simulink model "r2_b16a4x64f"  (R2012b)
settings: Solver=VariableStepDiscrete  SolverMode=SingleTasking  StartTime=0.0  StopTime=1  RelTol=1e-3
undefined symbols (not defined in the file): fft_stages, n_bits_ants, n_bits_xengs
libraries: xbsIndex_r4 x26846, casper_library_misc x230, xbsReplacements_r4 x24, casper_library_delays x8, xps_library x5, casper_library_communications x4
(part 46 of 227)

== system r2_b16a4x64f/sys2/Delay89 ==
  d : Inport
  Register0 : xbsIndex_r4/Register  init=0  rst=off  en=off  dbl_ovrd=off  block_type=register
      settings: block_version=11.4
  Register1 : xbsIndex_r4/Register  init=0  rst=off  en=off  dbl_ovrd=off  block_type=register
  q : Outport
  wires:
  Register0/1 -> Register1/1
  d/1 -> Register0/1
  Register1/1 -> q/1

== system r2_b16a4x64f/sys2/Delay9 ==
  d : Inport
  Register0 : xbsIndex_r4/Register  init=0  rst=off  en=off  dbl_ovrd=off  block_type=register
      settings: block_version=11.4
  Register1 : xbsIndex_r4/Register  init=0  rst=off  en=off  dbl_ovrd=off  block_type=register
  q : Outport
  wires:
  Register0/1 -> Register1/1
  d/1 -> Register0/1
  Register1/1 -> q/1

== system r2_b16a4x64f/sys2/bf ==
  synci : Inport
  di : Inport  Port=2
  deni : Inport  Port=3
  badi : Inport  Port=4
  timei : Inport  Port=5
  misci : Inport  Port=6
  beng_id : Inport  Port=7
  Delay1 : xbsIndex_r4/Delay  rst=off  infoeditControl=Selection of Reset will increase slice count due to use of real FFs and instead of SRLs  en=off  latency=1  dbl_ovrd=off  reg_retiming=on  block_type=delay
  Delay2 : xbsIndex_r4/Delay  rst=off  infoeditControl=Selection of Reset will increase slice count due to use of real FFs and instead of SRLs  en=off  latency=1  dbl_ovrd=off  reg_retiming=on  block_type=delay
  Relational : xbsIndex_r4/Relational  mode=a=b  en=off  latency=1  dbl_ovrd=off  block_type=relational
  Slice : xbsIndex_r4/Slice  nbits=bfpga_bits  boolean_output=off  mode=Lower Bit Location + Width  bit1=0  base1=MSB of Input  bit0=0  base0=LSB of Input  dbl_ovrd=off  block_type=slice
  fbf : Subsystem  mask(fbf){beng_bits=beng_bits, ant_bits=ant_bits, polarisation_bits=polarisation_bits, freq_bits=freq_bits, stack_bits=stack_bits, n_bits_in=n_bits_in, bin_pt_in=bin_pt_in, timestamp_bits=timestamp_bits, n_bits_norm=n_bits_norm, bin_pt_norm=bin_pt_norm, n_bits_combine=n_bits_combine, n_bits_requant=n_bits_requant, bin_pt_requant=bin_pt_requant, bram_latency=bram_latency, add_latency=add_latency, mult_latency=mult_latency, beam_bits=beam_bits, n_bits_out=n_bits_out, bin_pt_out=bin_pt_out, conv_latency=conv_latency, output_enabled=off}
      mask prompts: beng_bits "b-engines (2^?)"; ant_bits "antennas (2^?)"; polarisation_bits "polarisations (2^?)"; freq_bits "frequencies (2^?)"; stack_bits "stacking factor (2^?)"; n_bits_in "data bits in"; bin_pt_in "binary point in"; timestamp_bits "timestamp size (bits)"; n_bits_norm "calibration factor data bits"; bin_pt_norm "calibration factor binary point"; n_bits_combine "antenna combination output bit width"; n_bits_requant "requantization factor bit width"; bin_pt_requant "requantization factor binary point"; bram_latency "bram latency"; add_latency "add latency"; beam_bits "beams (2^?)"; n_bits_out "data bits out"; bin_pt_out "binary point out"; conv_latency "convert latency"; output_enabled "output enabled by default?"
      mask help:
      | Frequency domain beamformer
      |
      | b-engines: number of b-engines in system (same as x-engines)
      | stacking factor: the number of consecutive time samples in a data block
      | calibration factor: the complex factor multiplied with the incoming data.
      | The complex value is unique to each beam, input and frequency.
      | Requantization factor: real factor multiplied with the output data before
      | quantization. The value is unique to each beam and frequency.
      | beams: the number of beams per polarisation
      | ouput enabled by default: can be useful for simulation
      mask init:
      | set_param([gcb,'/filter'], ...
      |     'output_enabled', output_enabled);
      mask Help:
      | Accepts the same channelised data as the CASPER FX correlator x-engine core.
      | Polarisations appear in order in different beams. (for polarisation (0,1), 0 in [0,2...], 1 in [1,3...]).
      | TODO: beam steering.
      | TODO: Stokes output.
      | TODO: accumulation.
  synco : Outport
  do : Outport  Port=2
  deno : Outport  Port=3
  timeo : Outport  Port=4
  misco : Outport  Port=5
  value_out_bw : Outport  Port=6
  value_out_quant : Outport  Port=7
  value_out_filt : Outport  Port=8
  wires:
  fbf/3(deno) -> deno/1
  di/1 -> fbf/2(di)
  timei/1 -> fbf/5(timei)
  fbf/1(synco) -> synco/1
  [bf_stream] -> Delay2/1
  fbf/2(do) -> do/1
  misci/1 -> fbf/6(misci)
  synci/1 -> fbf/1(synci)
  deni/1 -> fbf/3(deni)
  [bf_antenna] -> Delay1/1
  badi/1 -> fbf/4(badi)
  fbf/4(timeo) -> timeo/1
  fbf/5(misco) -> misco/1
  fbf/6(bw_value_out) -> value_out_bw/1
  beng_id/1 -> Slice/1
  [bf_beng] -> Relational/2
  Slice/1 -> Relational/1
  Relational/1 -> fbf/9(ld_wr_en)
  Delay1/1 -> fbf/7(ld_antenna)
  Delay2/1 -> fbf/8(ld_stream)
  fbf/7(quant_value_out) -> value_out_quant/1
  fbf/8(filter_value_out) -> value_out_filt/1

== system r2_b16a4x64f/sys2/bus_expand1 ==
  bus_in : Inport
  reinterpret1 : xbsIndex_r4/Reinterpret  force_arith_type=on  arith_type=Unsigned  force_bin_pt=on  bin_pt=0  block_type=reinterpret
      settings: infoedit="Changes signal type without altering the binary representation.   You can changed the signal between signed and unsigned, and relocate the binary point.<br><br>Hardware notes: In hardware this block costs nothing.<br><br>Example:  Suppose the input is 6 bits wide, signed, with 2 fractional bits, and the output is forced to unsigned with 0 fractional bits.  Then an input of -2.0 (1110.00 in binary 2's complement) becomes an output of 56 (111000 in binary)."
  reinterpret3 : xbsIndex_r4/Reinterpret  force_arith_type=on  arith_type=Unsigned  force_bin_pt=on  bin_pt=0  block_type=reinterpret
  slice1 : xbsIndex_r4/Slice  nbits=32  boolean_output=off  mode=Upper Bit Location + Width  bit1=-28  base1=MSB of Input  bit0=0  base0=LSB of Input  dbl_ovrd=off  block_type=slice
  slice2 : xbsIndex_r4/Slice  nbits=1  boolean_output=on  mode=Upper Bit Location + Width  bit1=-27  base1=MSB of Input  bit0=0  base0=LSB of Input  dbl_ovrd=off  block_type=slice
  slice3 : xbsIndex_r4/Slice  nbits=27  boolean_output=off  mode=Upper Bit Location + Width  bit1=0  base1=MSB of Input  bit0=0  base0=LSB of Input  dbl_ovrd=off  block_type=slice
  msb_out3 : Outport
  out2 : Outport  Port=2
  lsb_out1 : Outport  Port=3
  wires:
  bus_in/1 -> slice3/1, slice2/1, slice1/1
  slice3/1 -> reinterpret3/1
  reinterpret3/1 -> msb_out3/1
  slice2/1 -> out2/1
  slice1/1 -> reinterpret1/1
  reinterpret1/1 -> lsb_out1/1

== system r2_b16a4x64f/sys2/bus_expand2 ==
  bus_in : Inport
  reinterpret1 : xbsIndex_r4/Reinterpret  force_arith_type=on  arith_type=Unsigned  force_bin_pt=on  bin_pt=0  block_type=reinterpret
  reinterpret2 : xbsIndex_r4/Reinterpret  force_arith_type=on  arith_type=Unsigned  force_bin_pt=on  bin_pt=0  block_type=reinterpret
  slice1 : xbsIndex_r4/Slice  nbits=19  boolean_output=off  mode=Upper Bit Location + Width  bit1=-27  base1=MSB of Input  bit0=0  base0=LSB of Input  dbl_ovrd=off  block_type=slice
  slice2 : xbsIndex_r4/Slice  nbits=27  boolean_output=off  mode=Upper Bit Location + Width  bit1=0  base1=MSB of Input  bit0=0  base0=LSB of Input  dbl_ovrd=off  block_type=slice
  msb_out2 : Outport
  lsb_out1 : Outport  Port=2
  wires:
  bus_in/1 -> slice2/1, slice1/1
  slice2/1 -> reinterpret2/1
  reinterpret2/1 -> msb_out2/1
  slice1/1 -> reinterpret1/1
  reinterpret1/1 -> lsb_out1/1

== system r2_b16a4x64f/sys2/bus_expand20 ==
  bus_in : Inport
  reinterpret1 : xbsIndex_r4/Reinterpret  force_arith_type=on  arith_type=Unsigned  force_bin_pt=on  bin_pt=0  block_type=reinterpret
      settings: infoedit="Changes signal type without altering the binary representation.   You can changed the signal between signed and unsigned, and relocate the binary point.<br><br>Hardware notes: In hardware this block costs nothing.<br><br>Example:  Suppose the input is 6 bits wide, signed, with 2 fractional bits, and the output is forced to unsigned with 0 fractional bits.  Then an input of -2.0 (1110.00 in binary 2's complement) becomes an output of 56 (111000 in binary)."
  reinterpret2 : xbsIndex_r4/Reinterpret  force_arith_type=on  arith_type=Unsigned  force_bin_pt=on  bin_pt=0  block_type=reinterpret
      settings: infoedit="Changes signal type without altering the binary representation.   You can changed the signal between signed and unsigned, and relocate the binary point.<br><br>Hardware notes: In hardware this block costs nothing.<br><br>Example:  Suppose the input is 6 bits wide, signed, with 2 fractional bits, and the output is forced to unsigned with 0 fractional bits.  Then an input of -2.0 (1110.00 in binary 2's complement) becomes an output of 56 (111000 in binary)."
  slice1 : xbsIndex_r4/Slice  nbits=19  boolean_output=off  mode=Upper Bit Location + Width  bit1=-33  base1=MSB of Input  bit0=0  base0=LSB of Input  dbl_ovrd=off  block_type=slice
  slice2 : xbsIndex_r4/Slice  nbits=33  boolean_output=off  mode=Upper Bit Location + Width  bit1=0  base1=MSB of Input  bit0=0  base0=LSB of Input  dbl_ovrd=off  block_type=slice
  msb_out2 : Outport
  lsb_out1 : Outport  Port=2
  wires:
  bus_in/1 -> slice2/1, slice1/1
  slice2/1 -> reinterpret2/1
  reinterpret2/1 -> msb_out2/1
  slice1/1 -> reinterpret1/1
  reinterpret1/1 -> lsb_out1/1

== system r2_b16a4x64f/sys2/bus_expand3 ==
  bus_in : Inport
  slice1 : xbsIndex_r4/Slice  nbits=1  boolean_output=on  mode=Upper Bit Location + Width  bit1=-5  base1=MSB of Input  bit0=0  base0=LSB of Input  dbl_ovrd=off  block_type=slice
  slice2 : xbsIndex_r4/Slice  nbits=1  boolean_output=on  mode=Upper Bit Location + Width  bit1=-4  base1=MSB of Input  bit0=0  base0=LSB of Input  dbl_ovrd=off  block_type=slice
  slice3 : xbsIndex_r4/Slice  nbits=1  boolean_output=on  mode=Upper Bit Location + Width  bit1=-3  base1=MSB of Input  bit0=0  base0=LSB of Input  dbl_ovrd=off  block_type=slice
  slice4 : xbsIndex_r4/Slice  nbits=1  boolean_output=on  mode=Upper Bit Location + Width  bit1=-2  base1=MSB of Input  bit0=0  base0=LSB of Input  dbl_ovrd=off  block_type=slice
  slice5 : xbsIndex_r4/Slice  nbits=1  boolean_output=on  mode=Upper Bit Location + Width  bit1=-1  base1=MSB of Input  bit0=0  base0=LSB of Input  dbl_ovrd=off  block_type=slice
  slice6 : xbsIndex_r4/Slice  nbits=1  boolean_output=on  mode=Upper Bit Location + Width  bit1=0  base1=MSB of Input  bit0=0  base0=LSB of Input  dbl_ovrd=off  block_type=slice
  msb_out6 : Outport
  out5 : Outport  Port=2
  out4 : Outport  Port=3
  out3 : Outport  Port=4
  out2 : Outport  Port=5
  lsb_out1 : Outport  Port=6
  wires:
  bus_in/1 -> slice6/1, slice5/1, slice4/1, slice3/1, slice2/1, slice1/1
  slice6/1 -> msb_out6/1
  slice5/1 -> out5/1
  slice4/1 -> out4/1
  slice3/1 -> out3/1
  slice2/1 -> out2/1
  slice1/1 -> lsb_out1/1

== system r2_b16a4x64f/sys2/bus_relational ==
  a : Inport
  b : Inport  Port=2
  a_debus : Subsystem  AncestorBlock=casper_library_flow_control/bus_expand  mask(bus_expand){mode=divisions of arbitrary size, outputNum=1, outputWidth=[1  1  1  1  1  1  1  1  1  1  1  1  1  1  1  1  1  1  1], outputBinaryPt=[0  0  0  0  0  0  0  0  0  0  0  0  0  0  0  0  0  0  0], outputArithmeticType=[0  0  0  0  0  0  0  0  0  0  0  0  0  0  0  0  0  0  0], show_format=on, outputToWorkspace=off, variablePrefix=, outputToModelAsWell=on}
      mask prompts: outputNum "Number of outputs:"; outputWidth "Output width [msb ... lsb]:"; outputBinaryPt "Output binary point position [msb ... lsb]:"; outputArithmeticType "Output arithmetic type (ufix=0, fix=1, bool=2) [msb ... lsb]:"; show_format "Print format string?"; outputToWorkspace "Output to workspace?"; variablePrefix "Variable name prefix:"; outputToModelAsWell "Output to model as well?"
      mask help:
      | Expands a 'bus' made using a bus_create or Xilinx
      | concat block.
      | The input will be divided into the specified number
      | of outputs with the specified arithmetic types.
      | Divisions are made from most significant bit.
      mask init: same as r2_b16a4x64f/bus_expand
      settings: AttributesFormatString=19 outputs: uf1.0,uf1.0,uf1.0,uf1.0,uf1.0,uf1.0,uf1.0,uf1.0,uf1.0,uf1.0,uf1.0,uf1.0,uf1.0,uf1.0,uf1.0,uf1.0,uf1.0,uf1.0,uf1.0,
      mask TypeOptions mode: divisions of equal size | divisions of arbitrary size
      mask Callback mode: bus_expand_callback();
      mask Callback outputWidth: bus_expand_callback();
      mask Callback outputToWorkspace: bus_expand_callback();
  b_debus : Subsystem  AncestorBlock=casper_library_flow_control/bus_expand  mask(bus_expand){mode=divisions of arbitrary size, outputNum=1, outputWidth=[1  1  1  1  1  1  1  1  1  1  1  1  1  1  1  1  1  1  1], outputBinaryPt=[0  0  0  0  0  0  0  0  0  0  0  0  0  0  0  0  0  0  0], outputArithmeticType=[0  0  0  0  0  0  0  0  0  0  0  0  0  0  0  0  0  0  0], show_format=on, outputToWorkspace=off, variablePrefix=, outputToModelAsWell=on}
      mask prompts: outputNum "Number of outputs:"; outputWidth "Output width [msb ... lsb]:"; outputBinaryPt "Output binary point position [msb ... lsb]:"; outputArithmeticType "Output arithmetic type (ufix=0, fix=1, bool=2) [msb ... lsb]:"; show_format "Print format string?"; outputToWorkspace "Output to workspace?"; variablePrefix "Variable name prefix:"; outputToModelAsWell "Output to model as well?"
      mask help:
      | Expands a 'bus' made using a bus_create or Xilinx
      | concat block.
      | The input will be divided into the specified number
      | of outputs with the specified arithmetic types.
      | Divisions are made from most significant bit.
      mask init: same as r2_b16a4x64f/bus_expand
      settings: AttributesFormatString=19 outputs: uf1.0,uf1.0,uf1.0,uf1.0,uf1.0,uf1.0,uf1.0,uf1.0,uf1.0,uf1.0,uf1.0,uf1.0,uf1.0,uf1.0,uf1.0,uf1.0,uf1.0,uf1.0,uf1.0,
      mask TypeOptions mode: divisions of equal size | divisions of arbitrary size
      mask Callback mode: bus_expand_callback();
      mask Callback outputWidth: bus_expand_callback();
      mask Callback outputToWorkspace: bus_expand_callback();
  bussify : Subsystem  AncestorBlock=casper_library_flow_control/bus_create  mask(bus_create){inputNum=19}
      mask prompts: inputNum "Number of inputs:"
      mask init:
      | bus_create_init(gcb,...
      |     'inputNum', inputNum);
  relational{1..19} (19 alike) : xbsIndex_r4/Relational  mode=a!=b  en=off  latency=0  dbl_ovrd=off  block_type=relational
  a!=b : Outport
  wires:
  a/1 -> a_debus/1(bus_in)
  b/1 -> b_debus/1(bus_in)
  a_debus/1(msb_out19) -> relational1/1
  b_debus/1(msb_out19) -> relational1/2
  a_debus/2(out18) -> relational2/1
  b_debus/2(out18) -> relational2/2
  a_debus/3(out17) -> relational3/1
  b_debus/3(out17) -> relational3/2
  a_debus/4(out16) -> relational4/1
  b_debus/4(out16) -> relational4/2
  a_debus/5(out15) -> relational5/1
  b_debus/5(out15) -> relational5/2
  a_debus/6(out14) -> relational6/1
  b_debus/6(out14) -> relational6/2
  a_debus/7(out13) -> relational7/1
  b_debus/7(out13) -> relational7/2
  a_debus/8(out12) -> relational8/1
  b_debus/8(out12) -> relational8/2
  a_debus/9(out11) -> relational9/1
  b_debus/9(out11) -> relational9/2
  a_debus/10(out10) -> relational10/1
  b_debus/10(out10) -> relational10/2
  a_debus/11(out9) -> relational11/1
  b_debus/11(out9) -> relational11/2
  a_debus/12(out8) -> relational12/1
  b_debus/12(out8) -> relational12/2
  a_debus/13(out7) -> relational13/1
  b_debus/13(out7) -> relational13/2
  a_debus/14(out6) -> relational14/1
  b_debus/14(out6) -> relational14/2
  a_debus/15(out5) -> relational15/1
  b_debus/15(out5) -> relational15/2
  a_debus/16(out4) -> relational16/1
  b_debus/16(out4) -> relational16/2
  a_debus/17(out3) -> relational17/1
  b_debus/17(out3) -> relational17/2
  a_debus/18(out2) -> relational18/1
  b_debus/18(out2) -> relational18/2
  a_debus/19(lsb_out1) -> relational19/1
  b_debus/19(lsb_out1) -> relational19/2
  relational1/1 -> bussify/1(in1)
  relational2/1 -> bussify/2(in2)
  relational3/1 -> bussify/3(in3)
  relational4/1 -> bussify/4(in4)
  relational5/1 -> bussify/5(in5)
  relational6/1 -> bussify/6(in6)
  relational7/1 -> bussify/7(in7)
  relational8/1 -> bussify/8(in8)
  relational9/1 -> bussify/9(in9)
  relational10/1 -> bussify/10(in10)
  relational11/1 -> bussify/11(in11)
  relational12/1 -> bussify/12(in12)
  relational13/1 -> bussify/13(in13)
  relational14/1 -> bussify/14(in14)
  relational15/1 -> bussify/15(in15)
  relational16/1 -> bussify/16(in16)
  relational17/1 -> bussify/17(in17)
  relational18/1 -> bussify/18(in18)
  relational19/1 -> bussify/19(in19)
  bussify/1(bus_out) -> a!=b/1

== system r2_b16a4x64f/sys2/flag_mux ==
  note: will load flag on current or
      | next valid data cycle
  tvg_en : Inport
  ld_val : Inport  Port=2
  en : Inport  Port=3
  misci : Inport  Port=4
  flag : Inport  Port=5
  tvg_flag : Inport  Port=6
  Constant30 : xbsIndex_r4/Constant  const=0  gui_display_data_type=Fixed-point  arith_type=Unsigned  n_bits=n_bits  bin_pt=0  preci_type=Single  exp_width=8  frac_width=24  explicit_period=on  period=1  equ=P=C  opselect=C  inp2=PCIN>>17  opr=+  inp1=P  carry=CIN  dbl_ovrd=off  block_type=constant
  Delay{1,98,100..102,104,106..107} (8 alike) : xbsIndex_r4/Delay  rst=off  infoeditControl=Selection of Reset will increase slice count due to use of real FFs and instead of SRLs  en=off  latency=1  dbl_ovrd=off  reg_retiming=on  block_type=delay
  Logical : xbsIndex_r4/Logical  logical_function=AND  inputs=2  en=off  latency=0  precision=Full  arith_type=Unsigned  n_bits=16  bin_pt=0  align_bp=on  dbl_ovrd=off  block_type=logical
  Mux2 : xbsIndex_r4/Mux  inputs=2  en=off  latency=1  precision=Full  arith_type=Unsigned  n_bits=16  bin_pt=14  quantization=Truncate  overflow=Wrap  dbl_ovrd=off  block_type=mux
  Mux3 : xbsIndex_r4/Mux  inputs=2  en=off  latency=1  precision=Full  arith_type=Unsigned  n_bits=16  bin_pt=14  quantization=Truncate  overflow=Wrap  dbl_ovrd=off  block_type=mux
  Register : xbsIndex_r4/Register  init=0  rst=on  en=on  dbl_ovrd=off  block_type=register
  dvalid : Outport
  misco : Outport  Port=2
  flags_out : Outport  Port=3
  wires:
  Delay107/1 -> Mux3/2
  Delay104/1 -> Delay102/1
  Delay106/1 -> Delay100/1
  Constant30/1 -> Mux2/2
  tvg_flag/1 -> Mux2/3
  Delay101/1 -> Delay104/1, Logical/1
  Mux2/1 -> Mux3/3
  Register/1 -> Logical/2
  ld_val/1 -> Register/1, Register/3
  Logical/1 -> Register/2, Mux2/1
  flag/1 -> Delay1/1
  en/1 -> Delay101/1
  misci/1 -> Delay98/1
  tvg_en/1 -> Mux3/1
  Delay98/1 -> Delay106/1
  Delay100/1 -> misco/1
  Mux3/1 -> flags_out/1
  Delay102/1 -> dvalid/1
  Delay1/1 -> Delay107/1

== system r2_b16a4x64f/sys2/flags ==
  flagsi : Inport
  Concat : xbsIndex_r4/Concat  num_inputs=4+1+11+1+5+1+4  dbl_ovrd=off  block_type=concat
  Constant : xbsIndex_r4/Constant  const=0  gui_display_data_type=Fixed-point  arith_type=Unsigned  n_bits=16-(3)  bin_pt=0  preci_type=Single  exp_width=8  frac_width=24  explicit_period=on  period=1  equ=P=C  opselect=C  inp2=PCIN>>17  opr=+  inp1=P  carry=CIN  dbl_ovrd=off  block_type=constant
  Constant1 : xbsIndex_r4/Constant  const=0  gui_display_data_type=Fixed-point  arith_type=Unsigned  n_bits=8-(4)  bin_pt=0  preci_type=Single  exp_width=8  frac_width=24  explicit_period=on  period=1  equ=P=C  opselect=C  inp2=PCIN>>17  opr=+  inp1=P  carry=CIN  dbl_ovrd=off  block_type=constant
  Constant2 : xbsIndex_r4/Constant  const=0  gui_display_data_type=Fixed-point  arith_type=Unsigned  n_bits=16-(11)  bin_pt=0  preci_type=Single  exp_width=8  frac_width=24  explicit_period=on  period=1  equ=P=C  opselect=C  inp2=PCIN>>17  opr=+  inp1=P  carry=CIN  dbl_ovrd=off  block_type=constant
  Constant3 : xbsIndex_r4/Constant  const=0  gui_display_data_type=Fixed-point  arith_type=Unsigned  n_bits=8-(5)  bin_pt=0  preci_type=Single  exp_width=8  frac_width=24  explicit_period=on  period=1  equ=P=C  opselect=C  inp2=PCIN>>17  opr=+  inp1=P  carry=CIN  dbl_ovrd=off  block_type=constant
  Logical : xbsIndex_r4/Logical  logical_function=OR  inputs=7  en=off  latency=0  precision=Full  arith_type=Unsigned  n_bits=16  bin_pt=0  align_bp=on  dbl_ovrd=off  block_type=logical
  Logical{1..4} (4 alike) : xbsIndex_r4/Logical  logical_function=OR  inputs=2  en=off  latency=0  precision=Full  arith_type=Unsigned  n_bits=16  bin_pt=0  align_bp=on  dbl_ovrd=off  block_type=logical
  bus_expand : Subsystem  AncestorBlock=casper_library_flow_control/bus_expand  mask(bus_expand){mode=divisions of arbitrary size, outputNum=1, outputWidth=[5 11 4], outputBinaryPt=[0 0 0], outputArithmeticType=[0 0 0], show_format=off, outputToWorkspace=off, variablePrefix=out, outputToModelAsWell=on}
      mask prompts: outputNum "Number of outputs:"; outputWidth "Output width [msb ... lsb]:"; outputBinaryPt "Output binary point position [msb ... lsb]:"; outputArithmeticType "Output arithmetic type (ufix=0, fix=1, bool=2) [msb ... lsb]:"; show_format "Print format string?"; outputToWorkspace "Output to workspace?"; variablePrefix "Variable name prefix:"; outputToModelAsWell "Output to model as well?"
      mask help:
      | Expands a 'bus' made using a bus_create or Xilinx
      | concat block.
      | The input will be divided into the specified number
      | of outputs with the specified arithmetic types.
      | Divisions are made from most significant bit.
      mask init: same as r2_b16a4x64f/bus_expand
      settings: AttributesFormatString=3 outputs
      mask TypeOptions mode: divisions of equal size | divisions of arbitrary size
      mask Callback mode: bus_expand_callback();
      mask Callback outputWidth: bus_expand_callback();
      mask Callback outputToWorkspace: bus_expand_callback();
  bus_expand1 : Subsystem  AncestorBlock=casper_library_flow_control/bus_expand  mask(bus_expand){mode=divisions of arbitrary size, outputNum=1, outputWidth=[1 1 1 1], outputBinaryPt=[0 0 0 0], outputArithmeticType=[0 0 0 0], show_format=off, outputToWorkspace=off, variablePrefix=out, outputToModelAsWell=on}
      mask prompts: outputNum "Number of outputs:"; outputWidth "Output width [msb ... lsb]:"; outputBinaryPt "Output binary point position [msb ... lsb]:"; outputArithmeticType "Output arithmetic type (ufix=0, fix=1, bool=2) [msb ... lsb]:"; show_format "Print format string?"; outputToWorkspace "Output to workspace?"; variablePrefix "Variable name prefix:"; outputToModelAsWell "Output to model as well?"
      mask help:
      | Expands a 'bus' made using a bus_create or Xilinx
      | concat block.
      | The input will be divided into the specified number
      | of outputs with the specified arithmetic types.
      | Divisions are made from most significant bit.
      mask init: same as r2_b16a4x64f/bus_expand
      settings: AttributesFormatString=4 outputs
      mask TypeOptions mode: divisions of equal size | divisions of arbitrary size
      mask Callback mode: bus_expand_callback();
      mask Callback outputWidth: bus_expand_callback();
      mask Callback outputToWorkspace: bus_expand_callback();
  bus_expand2 : Subsystem  AncestorBlock=casper_library_flow_control/bus_expand  mask(bus_expand){mode=divisions of arbitrary size, outputNum=1, outputWidth=[1 1 1 1 1 1 1 1 1 1 1], outputBinaryPt=[0 0 0 0 0 0 0 0 0 0 0], outputArithmeticType=[0 0 0 0 0 0 0 0 0 0 0], show_format=off, outputToWorkspace=off, variablePrefix=out, outputToModelAsWell=on}
      mask prompts: outputNum "Number of outputs:"; outputWidth "Output width [msb ... lsb]:"; outputBinaryPt "Output binary point position [msb ... lsb]:"; outputArithmeticType "Output arithmetic type (ufix=0, fix=1, bool=2) [msb ... lsb]:"; show_format "Print format string?"; outputToWorkspace "Output to workspace?"; variablePrefix "Variable name prefix:"; outputToModelAsWell "Output to model as well?"
      mask help:
      | Expands a 'bus' made using a bus_create or Xilinx
      | concat block.
      | The input will be divided into the specified number
      | of outputs with the specified arithmetic types.
      | Divisions are made from most significant bit.
      mask init: same as r2_b16a4x64f/bus_expand
      settings: AttributesFormatString=11 outputs
      mask TypeOptions mode: divisions of equal size | divisions of arbitrary size
      mask Callback mode: bus_expand_callback();
      mask Callback outputWidth: bus_expand_callback();
      mask Callback outputToWorkspace: bus_expand_callback();
  bus_expand3 : Subsystem  AncestorBlock=casper_library_flow_control/bus_expand  mask(bus_expand){mode=divisions of arbitrary size, outputNum=1, outputWidth=[1 1 1 1 1], outputBinaryPt=[0 0 0 0 0], outputArithmeticType=[0 0 0 0 0], show_format=off, outputToWorkspace=off, variablePrefix=out, outputToModelAsWell=on}
      mask prompts: outputNum "Number of outputs:"; outputWidth "Output width [msb ... lsb]:"; outputBinaryPt "Output binary point position [msb ... lsb]:"; outputArithmeticType "Output arithmetic type (ufix=0, fix=1, bool=2) [msb ... lsb]:"; show_format "Print format string?"; outputToWorkspace "Output to workspace?"; variablePrefix "Variable name prefix:"; outputToModelAsWell "Output to model as well?"
      mask help:
      | Expands a 'bus' made using a bus_create or Xilinx
      | concat block.
      | The input will be divided into the specified number
      | of outputs with the specified arithmetic types.
      | Divisions are made from most significant bit.
      mask init: same as r2_b16a4x64f/bus_expand
      settings: AttributesFormatString=5 outputs
      mask TypeOptions mode: divisions of equal size | divisions of arbitrary size
      mask Callback mode: bus_expand_callback();
      mask Callback outputWidth: bus_expand_callback();
      mask Callback outputToWorkspace: bus_expand_callback();
  flagso : Outport
  error : Outport  Port=2
  warning : Outport  Port=3
  wires:
  flagsi/1 -> bus_expand/1(bus_in)
  Concat/1 -> flagso/1
  bus_expand/3(lsb_out1) -> bus_expand1/1(bus_in)
  bus_expand1/4(lsb_out1) -> [noise_diode1]
  bus_expand/2(out2) -> bus_expand2/1(bus_in)
  bus_expand/1(msb_out3) -> bus_expand3/1(bus_in)
  bus_expand3/1(msb_out5) -> [vacc_error]
  bus_expand2/1(msb_out11) -> [qdr_parity_err0]
  bus_expand2/2(out10) -> [qdr_parity_err1]
  bus_expand2/3(out9) -> [pfb_or0]
  bus_expand2/4(out8) -> [pfb_or1]
  bus_expand3/4(out2) -> [discarding]
  bus_expand3/5(lsb_out1) -> [spead_error]
  bus_expand3/2(out4) -> [timed_out]
  bus_expand3/3(out3) -> [rcv_error]
  bus_expand2/11(lsb_out1) -> [f_spead_error]
  bus_expand2/10(out2) -> [f_fifo_of]
  bus_expand2/9(out3) -> [f_pkt_of]
  bus_expand2/8(out4) -> [f_discarding]
  bus_expand2/7(out5) -> [f_timed_out]
  bus_expand2/5(out7) -> [f_time_error]
  bus_expand2/6(out6) -> [f_rcv_error]
  bus_expand1/1(msb_out4) -> [adc_or0]
  bus_expand1/2(out3) -> [adc_or1]
  bus_expand1/3(out2) -> [noise_diode0]
  [adc_or0] -> Logical2/1
  [adc_or1] -> Logical2/2
  [pfb_or0] -> Logical3/1
  [pfb_or1] -> Logical3/2
  Logical2/1 -> Logical1/1
  Logical3/1 -> Logical1/2
  [noise_diode0] -> Logical4/1
  [noise_diode1] -> Logical4/2
  Constant/1 -> Concat/1
  Logical/1 -> error/1, Concat/2
  Logical1/1 -> warning/1, Concat/3
  Logical4/1 -> Concat/4
  [qdr_parity_err1] -> Concat/13
  [spead_error] -> Concat/10
  [qdr_parity_err0] -> Concat/12
  [f_pkt_of] -> Concat/20
  [discarding] -> Concat/9
  [f_rcv_error] -> Concat/17
  [f_timed_out] -> Concat/18
  [f_discarding] -> Concat/19
  [f_spead_error] -> Concat/22
  [noise_diode1] -> Concat/27
  [f_fifo_of] -> Concat/21
  [noise_diode0] -> Concat/26
  [f_time_error] -> Concat/16
  [rcv_error] -> Concat/8
  [timed_out] -> Concat/7
  [vacc_error] -> Concat/6
  [adc_or1] -> Concat/25
  [pfb_or0] -> Concat/14
  [adc_or0] -> Concat/24
  [pfb_or1] -> Concat/15
  Constant2/1 -> Concat/11
  Constant1/1 -> Concat/23
  Constant3/1 -> Concat/5
  [qdr_parity_err0] -> Logical/4
  [qdr_parity_err1] -> Logical/5
  [f_rcv_error] -> Logical/7
  [f_time_error] -> Logical/6
  [rcv_error] -> Logical/3
  [timed_out] -> Logical/2
  [vacc_error] -> Logical/1
